simulink model "Puzzolante10656823_Assign2_Ex2_Simscape"  (R2024b)
settings: Solver=VariableStepAuto  StartTime=0.0  StopTime=3 * T_orb  RelTol=1e-8  AbsTol=1e-9
undefined symbols (not defined in the file or in its folder): param
libraries: fl_lib x17, nesl_utility x7, ee_lib x1
settings Model: Creator=puzzo  LastModifiedBy=puzzo
settings SolverCC: AutoScaleAbsTol=off  AlgebraicLoopSolver=TrustRegion  MaxZcPerStep=1
settings DebuggingCC: AlgebraicLoopMsg=none  UnconnectedInputMsg=warning  UnconnectedOutputMsg=warning  UnconnectedLineMsg=warning  SymbolicDimsDataTypeCodeGenerationDiagnostic=none
settings ModelReferenceCC: EnableRefExpFcnMdlSchedulingChecks=on
settings SFSimCC: CustomCodeUndefinedFunction=UseInterfaceOnly
settings RTWCC: GPUComputeCapability=3.5  DLArmComputeVersion=19.05
settings SimscapeCC: SimscapeLogType=all  SimscapeLogSimulationStatistics=on  SimscapeLogDataHistory=10000

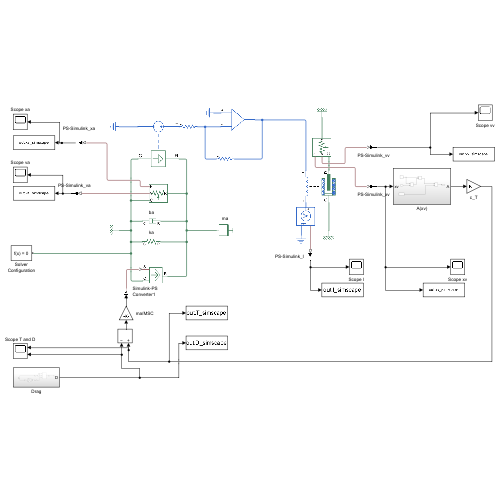
[thumbnail: Simulink's stored preview of the top-level diagram]
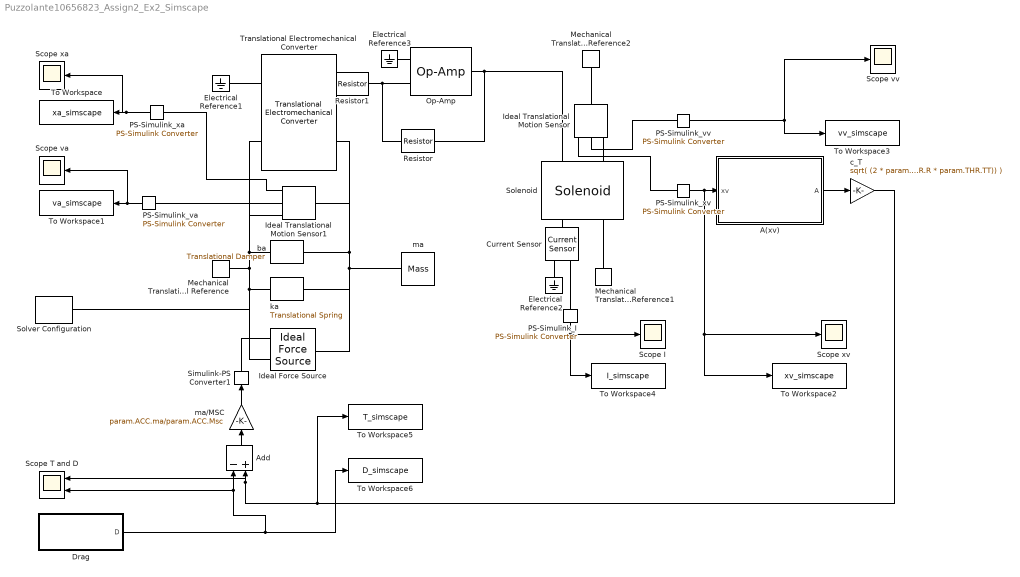
== system Puzzolante10656823_Assign2_Ex2_Simscape ==
  A(xv) : Subsystem
  Add : Sum  Inputs=-+
  Current Sensor : fl_lib/Electrical/Electrical Sensors/Current Sensor
  Drag : Subsystem
  Electrical Reference1 : fl_lib/Electrical/Electrical Elements/Electrical Reference
  Electrical Reference2 : fl_lib/Electrical/Electrical Elements/Electrical Reference
  Electrical Reference3 : fl_lib/Electrical/Electrical Elements/Electrical Reference
  Ideal Force Source : fl_lib/Mechanical/Mechanical Sources/Ideal Force Source
  Ideal Translational Motion Sensor : fl_lib/Mechanical/Mechanical Sensors/Ideal Translational Motion Sensor  reference=foundation.enum.MeasurementReference.difference  acceleration_port=false  velocity_port=true  position_port=true  offset=xv0 m
  Ideal Translational Motion Sensor1 : fl_lib/Mechanical/Mechanical Sensors/Ideal Translational Motion Sensor  reference=foundation.enum.MeasurementReference.difference  acceleration_port=false  velocity_port=true  position_port=true  offset=xa0 m
  Mechanical Translational Reference : fl_lib/Mechanical/Translational Elements/Mechanical Translational Reference
  Mechanical Translational Reference1 : fl_lib/Mechanical/Translational Elements/Mechanical Translational Reference
  Mechanical Translational Reference2 : fl_lib/Mechanical/Translational Elements/Mechanical Translational Reference
  Op-Amp : fl_lib/Electrical/Electrical Elements/Op-Amp  outI_specify=off  outI_priority=None  outI=0 A  outI_nominal_specify=off  outI_nominal_value=1  outI_nominal_unit=A
  PS-Simulink_I : nesl_utility/PS-Simulink Converter  PhysicalDomain=network_engine_domain  SubClassName=ps_output  LeftPortType=input  RightPortType=output  PseudoPeriodic=off  Frequencies=[]  VectorFormat=inherit  Unit=inherit  AffineConversion=off
  PS-Simulink_va : nesl_utility/PS-Simulink Converter  PhysicalDomain=network_engine_domain  SubClassName=ps_output  LeftPortType=input  RightPortType=output  PseudoPeriodic=off  Frequencies=[]  VectorFormat=inherit  Unit=inherit  AffineConversion=off
  PS-Simulink_vv : nesl_utility/PS-Simulink Converter  PhysicalDomain=network_engine_domain  SubClassName=ps_output  LeftPortType=input  RightPortType=output  PseudoPeriodic=off  Frequencies=[]  VectorFormat=inherit  Unit=inherit  AffineConversion=off
  "PS-Simulink_xa " : nesl_utility/PS-Simulink Converter  PhysicalDomain=network_engine_domain  SubClassName=ps_output  LeftPortType=input  RightPortType=output  PseudoPeriodic=off  Frequencies=[]  VectorFormat=inherit  Unit=inherit  AffineConversion=off
  PS-Simulink_xv : nesl_utility/PS-Simulink Converter  PhysicalDomain=network_engine_domain  SubClassName=ps_output  LeftPortType=input  RightPortType=output  PseudoPeriodic=off  Frequencies=[]  VectorFormat=inherit  Unit=inherit  AffineConversion=off
  Resistor : fl_lib/Electrical/Electrical Elements/Resistor  R=param.AMP.Rf Ohm  i_specify=off  i_priority=None  i=I0 A  i_nominal_specify=off  i_nominal_value=1  i_nominal_unit=A  v_specify=off  v_priority=None  v=0 V  v_nominal_specify=off  v_nominal_value=1  v_nominal_unit=V
  Resistor1 : fl_lib/Electrical/Electrical Elements/Resistor  R=param.AMP.Rin Ohm  i_specify=off  i_priority=None  i=0 A  i_nominal_specify=off  i_nominal_value=1  i_nominal_unit=A  v_specify=off  v_priority=None  v=0 V  v_nominal_specify=off  v_nominal_value=1  v_nominal_unit=V
  Scope I : Scope
  Scope T and D : Scope  NumInputPorts=2
  Scope va : Scope
  Scope vv : Scope
  Scope xa : Scope
  Scope xv : Scope
  Simulink-PS Converter1 : nesl_utility/Simulink-PS Converter  PhysicalDomain=network_engine_domain  SubClassName=ps_input  LeftPortType=input  RightPortType=output  PseudoPeriodic=off  Frequencies=[]  NoiseDistribution=none  NoiseParameters=[]  Unit=1  AffineConversion=off  FilteringAndDerivatives=provide  SimscapeFilterOrder=1  InputFilterTimeConstant=0.001  UdotUserProvided=0
  Solenoid : ee_lib/Electromechanical/Mechatronic Actuators/Solenoid  motionDirection=ee.enum.actuators.solenoidDirection.towards  F12=[9000 12] N  X12=[0 1e-4] m  Vdc=6e-4 V  Imax=0.1 A  K=param.SOLV.kv N/m  Xzero=param.SOLV.xv_max m  lam=param.SOLV.bv N*s/m  Mass=param.SOLV.mv kg  Xmax=1e-4 m  K_endstop=0.12*10^6 N/m  D_endstop=10^4 N*s/m  i_specify=on  i_priority=High  i=I0 A  i_nominal_specify=off  i_nominal_value=1  i_nominal_unit=A  x_specify=on  x_priority=High  x=xv0 m  x_nominal_specify=off  x_nominal_value=1  x_nominal_unit=mm  vel_specify=on  vel_priority=High  vel=vv0 m/s  vel_nominal_specify=off  vel_nominal_value=1  vel_nominal_unit=mm/s  F_specify=off  F_priority=None  F=0 N  F_nominal_specify=off  F_nominal_value=1  F_nominal_unit=N  v_L_specify=off  v_L_priority=None  v_L=0 V  v_L_nominal_specify=off  v_L_nominal_value=1  v_L_nominal_unit=V  magnetic_force_specify=off  magnetic_force_priority=None  magnetic_force=0 N  magnetic_force_nominal_specify=off  magnetic_force_nominal_value=1  magnetic_force_nominal_unit=N  alpha=3.93e-3 1/K  Tmeas=25 degC  thermal_mass=100 J/K  temperature_specify=off  temperature_priority=High  temperature=25 degC  temperature_nominal_specify=off  temperature_nominal_value=1  temperature_nominal_unit=degC  Q_specify=off  Q_priority=None  Q=0 W  Q_nominal_specify=off  Q_nominal_value=1  Q_nominal_unit=W
      settings: InternalSimscapePortConfiguration="{\"Bottom\":[],\"Left\":[{\"id\":\"p\",\"label\":\"+\",\"type\":\"foundation.electrical.electrical\"},{\"id\":\"R\",\"label\":\"R\",\"type\":\"foundation.mechanical.translational.translational\"}],\"Right\":[{\"id\":\"n\",\"label\":\"-\",\"type\":\"foundation.electrical.electrical\"},{\"id\":\"C\",\"label\":\"C\",\"type\":\"foundation.mechanical.translational.translational\"}],\"Top\":[]}"
  Solver Configuration : nesl_utility/Solver Configuration  PhysicalDomain=network_engine_domain  SubClassName=solver  LeftPortType=input  RightPortType=generic  Tones=[]  Harmonics=[]  SimulateNoise=off  Profile=off  UseLocalSampling=off  EnableSwitchedLinearOptims=on  FrequencyDomain=off  UseCCode=off  RelTol=0.001  AbsTol=1e-06  MinStep=1e-09  ToWorkspace=off  RevertToSquareIcSolve=off  NumHomotopyIterations=100  PhasorMode=off  PhasorModeNumHarmonics=1  ConsistencySolver=NEWTON_XTOL_AFTER_FTOL  IndexReductionMethod=DerivativeReplacement  DoDC=off  ResidualTolerance=1e-09  ConsistencyTolSource=GLOBAL  ConsistencyAbsTol=0.001  ConsistencyRelTol=0.001  ConsistencyTolFactor=0.01  UseLocalSolver=off  LocalSolverChoice=NE_BACKWARD_EULER_ADVANCER  ResolveIndetEquations=on  FunctionEvalNumThread=1  LocalSolverSampleTime=0.001  DoFixedCost=off  MaxNonlinIter=3  MaxModeIter=2  ComputeImpulses=off  ImpulseIterations=2  LinearAlgebra=auto  LinearAlgebraNumThread=0  EquationFormulation=NE_TIME_EF  DelaysMemoryBudget=1024  AutomaticFiltering=on  FilteringTimeConstant=0.001  PartitionStorageMethod=AS_NEEDED  PartitionMemoryBudget=1024  PartitionMethod=ROBUST  MultibodyUseLocalSolver=off  MultibodyLocalSolverChoice=ODE1  MultibodyLocalSolverSampleTime=0.001
  To Workspace : ToWorkspace  VariableName=xa_simscape  SaveFormat=Structure With Time  SampleTime=-1
  To Workspace1 : ToWorkspace  VariableName=va_simscape  SaveFormat=Structure With Time  SampleTime=-1
  To Workspace2 : ToWorkspace  VariableName=xv_simscape  SaveFormat=Structure With Time  SampleTime=-1
  To Workspace3 : ToWorkspace  VariableName=vv_simscape  SaveFormat=Structure With Time  SampleTime=-1
  To Workspace4 : ToWorkspace  VariableName=I_simscape  SaveFormat=Structure With Time  SampleTime=-1
  To Workspace5 : ToWorkspace  VariableName=T_simscape  SaveFormat=Structure With Time  SampleTime=-1
  To Workspace6 : ToWorkspace  VariableName=D_simscape  SaveFormat=Structure With Time  SampleTime=-1
  Translational Electromechanical Converter : fl_lib/Electrical/Electrical Elements/Translational Electromechanical Converter  K=param.ACC.Kacc V*s/m  i_specify=off  i_priority=None  i=I0 A  i_nominal_specify=off  i_nominal_value=1  i_nominal_unit=A  v_specify=off  v_priority=None  v=0 V  v_nominal_specify=off  v_nominal_value=1  v_nominal_unit=V  f_specify=off  f_priority=None  f=0 N  f_nominal_specify=off  f_nominal_value=1  f_nominal_unit=N  u_specify=on  u_priority=None  u=va0 m/s  u_nominal_specify=off  u_nominal_value=1  u_nominal_unit=m/s
      settings: InternalSimscapePortConfiguration="{\"Bottom\":[],\"Left\":[{\"id\":\"p\",\"label\":\"+\",\"type\":\"foundation.electrical.electrical\"},{\"id\":\"R\",\"label\":\"R\",\"type\":\"foundation.mechanical.translational.translational\"}],\"Right\":[{\"id\":\"n\",\"label\":\"-\",\"type\":\"foundation.electrical.electrical\"},{\"id\":\"C\",\"label\":\"C\",\"type\":\"foundation.mechanical.translational.translational\"}],\"Top\":[]}"
  ba : fl_lib/Mechanical/Translational Elements/Translational Damper  D=param.ACC.ba N*s/m  v_specify=on  v_priority=High  v=va0 m/s  v_nominal_specify=off  v_nominal_value=1  v_nominal_unit=m/s  f_specify=off  f_priority=None  f=0 N  f_nominal_specify=off  f_nominal_value=1  f_nominal_unit=N
  c_T : Gain  Gain=sqrt( (2 * param.THR.V * param.THR.q)/param.THR.mi ) * sqrt(param.THR.k * param.THR.pT * (2/(param.THR.k + 1))^((param.THR.k + 1)/(param.THR.k - 1)) * (param.THR.pT/(param.THR.R * param.THR.TT)) )
  ka : fl_lib/Mechanical/Translational Elements/Translational Spring  spr_rate=param.ACC.ka N/m  v_specify=on  v_priority=High  v=va0 m/s  v_nominal_specify=off  v_nominal_value=1  v_nominal_unit=m/s  f_specify=off  f_priority=None  f=0 N  f_nominal_specify=off  f_nominal_value=1  f_nominal_unit=N  x_specify=on  x_priority=High  x=xa0 m  x_nominal_specify=off  x_nominal_value=1  x_nominal_unit=m
  ma : fl_lib/Mechanical/Translational Elements/Mass  mass=param.ACC.ma kg  num_ports=foundation.enum.numPorts2.one  v_specify=on  v_priority=High  v=va0 m/s  v_nominal_specify=off  v_nominal_value=1  v_nominal_unit=m/s  f_specify=off  f_priority=None  f=0 N  f_nominal_specify=off  f_nominal_value=1  f_nominal_unit=N
  ma/MSC : Gain  Gain=param.ACC.ma/param.ACC.Msc
  wires:
  PS-Simulink_xv/1 -> Scope xv/1, To Workspace2/1, A(xv)/1(xv)
  A(xv)/1(A) -> c_T/1
  Drag/1(D) -> Add/1, Scope T and D/2, To Workspace6/1
  c_T/1 -> Scope T and D/1, Add/2, To Workspace5/1
  ma/MSC/1 -> Simulink-PS Converter1/1
  Add/1 -> ma/MSC/1
  PS-Simulink_vv/1 -> Scope vv/1, To Workspace3/1
  PS-Simulink_va/1 -> Scope va/1, To Workspace1/1
  "PS-Simulink_xa "/1 -> Scope xa/1, To Workspace/1
  PS-Simulink_I/1 -> Scope I/1, To Workspace4/1
  connections:
  Mechanical Translational Reference/LConn1 -- Solver Configuration/RConn1 -- Ideal Force Source/RConn2 -- ka/RConn1 -- Ideal Translational Motion Sensor1/RConn1 -- Translational Electromechanical Converter/RConn2 -- ba/RConn1
  ba/LConn1 -- Ideal Translational Motion Sensor1/LConn1 -- Translational Electromechanical Converter/LConn2 -- Ideal Force Source/LConn1 -- ka/LConn1 -- ma/LConn1
  Mechanical Translational Reference1/LConn1 -- Solenoid/RConn2
  PS-Simulink_xv/LConn1 -- Ideal Translational Motion Sensor/RConn3
  Ideal Force Source/RConn1 -- Simulink-PS Converter1/RConn1
  Translational Electromechanical Converter/RConn1 -- Electrical Reference1/LConn1
  Solenoid/LConn1 -- Resistor/RConn1 -- Op-Amp/RConn1
  Resistor/LConn1 -- Op-Amp/LConn2 -- Resistor1/RConn1
  PS-Simulink_vv/LConn1 -- Ideal Translational Motion Sensor/RConn2
  "PS-Simulink_xa "/LConn1 -- Ideal Translational Motion Sensor1/RConn3
  PS-Simulink_va/LConn1 -- Ideal Translational Motion Sensor1/RConn2
  PS-Simulink_I/LConn1 -- Current Sensor/RConn1
  Electrical Reference3/LConn1 -- Op-Amp/LConn1
  Resistor1/LConn1 -- Translational Electromechanical Converter/LConn1
  Current Sensor/LConn1 -- Solenoid/RConn1
  Current Sensor/RConn2 -- Electrical Reference2/LConn1
  Ideal Translational Motion Sensor/LConn1 -- Mechanical Translational Reference2/LConn1
  Ideal Translational Motion Sensor/RConn1 -- Solenoid/LConn2

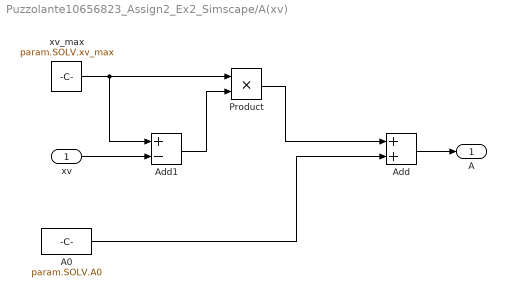
== system Puzzolante10656823_Assign2_Ex2_Simscape/A(xv) ==
  xv : Inport  Unit=m
  A0 : Constant  Value=param.SOLV.A0
  Add : Sum
  Add1 : Sum  Inputs=+-
  Product : Product
  xv_max : Constant  Value=param.SOLV.xv_max
  A : Outport
  wires:
  xv_max/1 -> Add1/1, Product/1
  xv/1 -> Add1/2
  Add1/1 -> Product/2
  Add/1 -> A/1
  A0/1 -> Add/2
  Product/1 -> Add/1

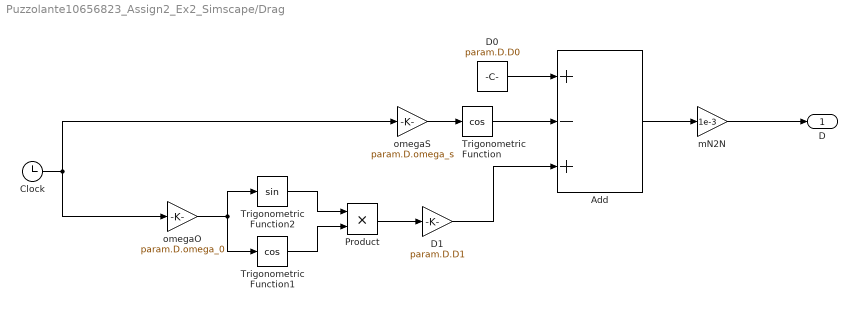
== system Puzzolante10656823_Assign2_Ex2_Simscape/Drag ==
  Add : Sum  Inputs=+-+
  Clock : Clock
  D0 : Constant  Value=param.D.D0
  D1 : Gain  Gain=param.D.D1
  Product : Product
  Trigonometric Function : Trigonometry  Operator=cos
  Trigonometric Function1 : Trigonometry  Operator=cos
  Trigonometric Function2 : Trigonometry
  mN2N : Gain  Gain=1e-3
  omegaO : Gain  Gain=param.D.omega_0
  omegaS : Gain  Gain=param.D.omega_s
  D : Outport
  wires:
  D0/1 -> Add/1
  omegaS/1 -> Trigonometric Function/1
  Trigonometric Function/1 -> Add/2
  omegaO/1 -> Trigonometric Function1/1, Trigonometric Function2/1
  Clock/1 -> omegaS/1, omegaO/1
  Trigonometric Function2/1 -> Product/1
  Trigonometric Function1/1 -> Product/2
  Product/1 -> D1/1
  D1/1 -> Add/3
  Add/1 -> mN2N/1
  mN2N/1 -> D/1
